simulink model "inverter_pwm"  (R2021a)
settings: Solver=VariableStepAuto  StartTime=0.0  StopTime=0.06  RelTol=1e-3
libraries: spsIGBTDiodeLib x12, simulink x5, spsCurrentMeasurementLib x3, spsDCVoltageSourceLib x3, spsSeriesRLCBranchLib x3, spsVoltageMeasurementLib x3, spspowerguiLib x1
settings Model: Creator=lenovo  LastModifiedBy=lenovo

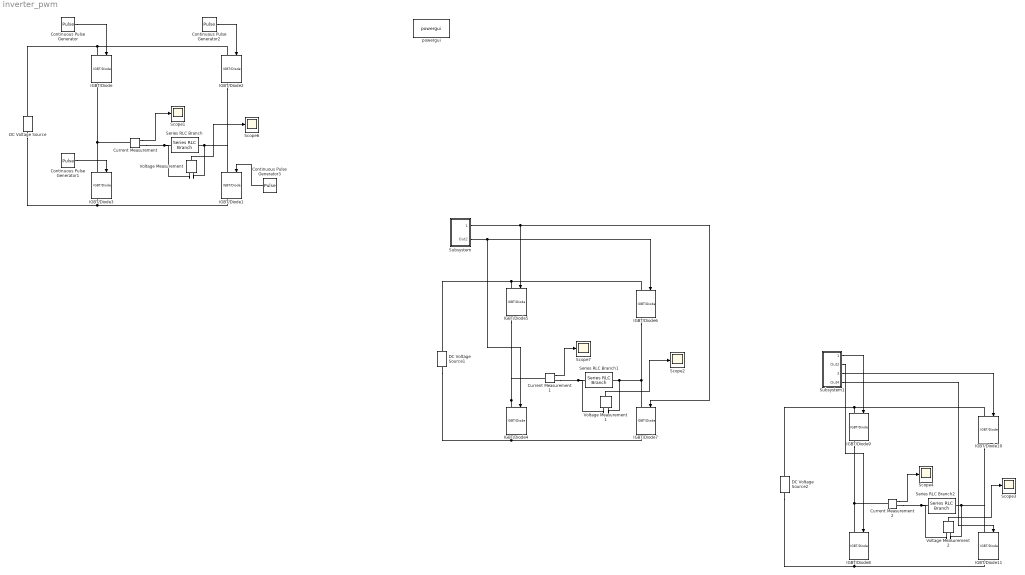
== system inverter_pwm ==
  Continuous Pulse Generator : DiscretePulseGenerator  PulseType=Time based  Period=1/50  PulseWidth=50
  Continuous Pulse Generator1 : DiscretePulseGenerator  PulseType=Time based  Period=1/50  PulseWidth=50  PhaseDelay=1/100
  Continuous Pulse Generator2 : DiscretePulseGenerator  PulseType=Time based  Period=1/50  PulseWidth=50  PhaseDelay=6/500
  Continuous Pulse Generator3 : DiscretePulseGenerator  PulseType=Time based  Period=1/50  PulseWidth=50  PhaseDelay=1/500
  Current Measurement : spsCurrentMeasurementLib/Current Measurement  PhasorSimulation=off  OutputType=Complex  PSBequivalent=0
  Current Measurement1 : spsCurrentMeasurementLib/Current Measurement  PhasorSimulation=off  OutputType=Complex  PSBequivalent=0
  Current Measurement2 : spsCurrentMeasurementLib/Current Measurement  PhasorSimulation=off  OutputType=Complex  PSBequivalent=0
  DC Voltage Source : spsDCVoltageSourceLib/DC Voltage Source  Amplitude=120  Measurements=None
  DC Voltage Source1 : spsDCVoltageSourceLib/DC Voltage Source  Amplitude=120  Measurements=None
  DC Voltage Source2 : spsDCVoltageSourceLib/DC Voltage Source  Amplitude=120  Measurements=None
  IGBT/Diode{,1..11} (12 alike) : spsIGBTDiodeLib/IGBT//Diode  Ron=1e-3  Rs=1e5  Cs=inf  Measurements=on
  Scope{1..4,6..7} (6 alike) : Scope
  Series RLC Branch : spsSeriesRLCBranchLib/Series RLC Branch  LConnTagsString=__new0  RConnTagsString=__new0  BranchType=RL  Resistance=1  Inductance=0.8  SetiL0=off  InitialCurrent=0  Capacitance=1e-6  Setx0=off  InitialVoltage=0  Measurements=None
  Series RLC Branch1 : spsSeriesRLCBranchLib/Series RLC Branch  LConnTagsString=__new0  RConnTagsString=__new0  BranchType=RL  Resistance=1  Inductance=0.1  SetiL0=off  InitialCurrent=0  Capacitance=1e-6  Setx0=off  InitialVoltage=0  Measurements=None
  Series RLC Branch2 : spsSeriesRLCBranchLib/Series RLC Branch  LConnTagsString=__new0  RConnTagsString=__new0  BranchType=RL  Resistance=1  Inductance=0.1  SetiL0=off  InitialCurrent=0  Capacitance=1e-6  Setx0=off  InitialVoltage=0  Measurements=None
  Subsystem : Subsystem
  Subsystem1 : Subsystem
  Voltage Measurement : spsVoltageMeasurementLib/Voltage Measurement  PhasorSimulation=off  OutputType=Complex  PSBequivalent=0
  Voltage Measurement1 : spsVoltageMeasurementLib/Voltage Measurement  PhasorSimulation=off  OutputType=Complex  PSBequivalent=0
  Voltage Measurement2 : spsVoltageMeasurementLib/Voltage Measurement  PhasorSimulation=off  OutputType=Complex  PSBequivalent=0
  powergui : spspowerguiLib/powergui  Priority=1  SimulationMode=Discrete  SampleTime=5e-6  frequency=60  Iterations=50  frequencyindice=0  Pbase=100e6  ErrMax=1e-4  UnitsV=kV  UnitsW=MW  buscounter=0  FunctionMessages=off  echomessages=off  EnableUseOfTLC=off  CurrentSourceSwitches=off  DisableSnubberDevices=off  DisableRonSwitches=off  DisableVfSwitches=off  DisplayEquations=off  AutomaticDiscreteSolvers=off  SolverType=Tustin/Backward Euler (TBE)  Interpol=off  ExternalGateDelay=off  methode=off  Ts=100  x0status=blocks  SPID=on  SwTol=0  HookPort=off  NonlinearTolerance=1e-4  nMaxIteration=100  ContinueOnMaxIteration=off  RestoreLinks=warning  ResistiveCurrentMeasurement=off  Frange=[0:2:500]  Ylog=off  Xlog=on  ShowGrid=off  save=off  variable=ZData  structure=0  ZoomFFT=off  StartTime=0.0  cycles=1  DisplayStyle=1  fundamental=60  FreqAxis=off  MaxFrequency=1000  frequencyindicesteady=1  RmsSteady=1  display=off
  wires:
  Continuous Pulse Generator/1 -> IGBT/Diode/1
  Continuous Pulse Generator2/1 -> IGBT/Diode2/1
  Continuous Pulse Generator1/1 -> IGBT/Diode3/1
  Continuous Pulse Generator3/1 -> IGBT/Diode1/1
  Voltage Measurement1/1 -> Scope2/1
  Subsystem/2(Out2) -> IGBT/Diode4/1, IGBT/Diode6/1
  Subsystem/1(" ") -> IGBT/Diode5/1, IGBT/Diode7/1
  Current Measurement1/1 -> Scope7/1
  Current Measurement2/1 -> Scope4/1
  Voltage Measurement2/1 -> Scope3/1
  Subsystem1/1(" ") -> IGBT/Diode9/1
  Subsystem1/3("   ") -> IGBT/Diode10/1
  Subsystem1/2(Out2) -> IGBT/Diode8/1
  Subsystem1/4(Out4) -> IGBT/Diode11/1
  Voltage Measurement/1 -> Scope6/1
  Current Measurement/1 -> Scope1/1
  connections:
  IGBT/Diode1/LConn1 -- IGBT/Diode2/RConn1 -- Voltage Measurement/LConn2 -- Series RLC Branch/RConn1
  Current Measurement/LConn1 -- IGBT/Diode3/LConn1 -- IGBT/Diode/RConn1
  DC Voltage Source/RConn1 -- IGBT/Diode2/LConn1 -- IGBT/Diode/LConn1
  DC Voltage Source/LConn1 -- IGBT/Diode3/RConn1 -- IGBT/Diode1/RConn1
  Current Measurement/RConn1 -- Voltage Measurement/LConn1 -- Series RLC Branch/LConn1
  IGBT/Diode4/RConn1 -- DC Voltage Source1/LConn1 -- IGBT/Diode7/RConn1
  Series RLC Branch1/LConn1 -- Current Measurement1/RConn1 -- Voltage Measurement1/LConn1
  IGBT/Diode6/RConn1 -- IGBT/Diode7/LConn1 -- Voltage Measurement1/LConn2 -- Series RLC Branch1/RConn1
  IGBT/Diode5/LConn1 -- DC Voltage Source1/RConn1 -- IGBT/Diode6/LConn1
  IGBT/Diode4/LConn1 -- IGBT/Diode5/RConn1 -- Current Measurement1/LConn1
  Series RLC Branch2/RConn1 -- IGBT/Diode10/RConn1 -- IGBT/Diode11/LConn1 -- Voltage Measurement2/LConn2
  IGBT/Diode11/RConn1 -- IGBT/Diode8/RConn1 -- DC Voltage Source2/LConn1
  Current Measurement2/LConn1 -- IGBT/Diode8/LConn1 -- IGBT/Diode9/RConn1
  IGBT/Diode10/LConn1 -- IGBT/Diode9/LConn1 -- DC Voltage Source2/RConn1
  Voltage Measurement2/LConn1 -- Series RLC Branch2/LConn1 -- Current Measurement2/RConn1

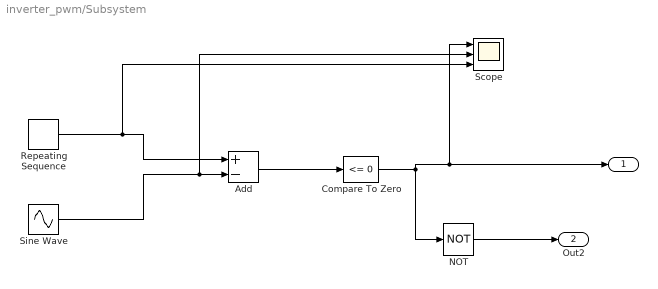
== system inverter_pwm/Subsystem ==
  Add : Sum  Inputs=+-
  Compare To Zero : simulink/Logic and Bit Operations/Compare To Zero  relop=<=  OutDataTypeStr=boolean
  NOT : Logic  Operator=NOT  IconShape=distinctive  AllPortsSameDT=off  OutDataTypeStr=boolean
  Repeating Sequence : simulink/Sources/Repeating Sequence  rep_seq_t=[0 0.00005 0.0001 0.00015 0.0002]  rep_seq_y=[0 1 0 -1 0]
  Scope : Scope  NumInputPorts=3
  Sine Wave : Sin  Amplitude=0.8  Frequency=314.159265  SampleTime=0  VectorParams1D=off
  " " : Outport
  Out2 : Outport  Port=2
  wires:
  Add/1 -> Compare To Zero/1
  Compare To Zero/1 -> Scope/1, " "/1, NOT/1
  Repeating Sequence/1 -> Scope/3, Add/1
  Sine Wave/1 -> Scope/2, Add/2
  NOT/1 -> Out2/1

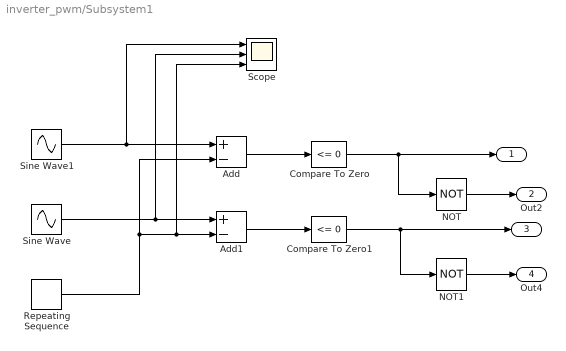
== system inverter_pwm/Subsystem1 ==
  Add : Sum  Inputs=+-
  Add1 : Sum  Inputs=+-
  Compare To Zero : simulink/Logic and Bit Operations/Compare To Zero  relop=<=  OutDataTypeStr=boolean
  Compare To Zero1 : simulink/Logic and Bit Operations/Compare To Zero  relop=<=  OutDataTypeStr=boolean
  NOT : Logic  Operator=NOT  IconShape=distinctive  AllPortsSameDT=off  OutDataTypeStr=boolean
  NOT1 : Logic  Operator=NOT  IconShape=distinctive  AllPortsSameDT=off  OutDataTypeStr=boolean
  Repeating Sequence : simulink/Sources/Repeating Sequence  rep_seq_t=[0 0.00005 0.0001 0.00015 0.0002]  rep_seq_y=[0 1 0 -1 0]
  Scope : Scope  NumInputPorts=3
  Sine Wave : Sin  Amplitude=0.8  Frequency=314.159265  SampleTime=0  VectorParams1D=off
  Sine Wave1 : Sin  Amplitude=-0.8  Frequency=314.159265  SampleTime=0  VectorParams1D=off
  " " : Outport
  Out2 : Outport  Port=2
  "   " : Outport  Port=3
  Out4 : Outport  Port=4
  wires:
  Repeating Sequence/1 -> Scope/3, Add1/2, Add/2
  NOT1/1 -> Out4/1
  Compare To Zero/1 -> " "/1, NOT/1
  Sine Wave1/1 -> Scope/1, Add/1
  Sine Wave/1 -> Scope/2, Add1/1
  Add/1 -> Compare To Zero/1
  Add1/1 -> Compare To Zero1/1
  NOT/1 -> Out2/1
  Compare To Zero1/1 -> "   "/1, NOT1/1
